simulink model "AFC_FFNN_trainbfg_15_15_15_15_Nor_July_15_RepFast"  (R2021a)
settings: Solver=ode15s  StartTime=0.0  StopTime=T  MaxStep=.01  RelTol=1e-3
undefined symbols (not defined in the file): AF_sensor_tol, fault_time, fuel_inj_tol, kappa_tol, MAF_sensor_tol, patch_sig, pump_tol, safe_patch_sig, sw, tau_ww_tol, x_gain, x_offset, y_gain, y_offset
libraries: neural x66, simulink x3
(part 3 of 3)

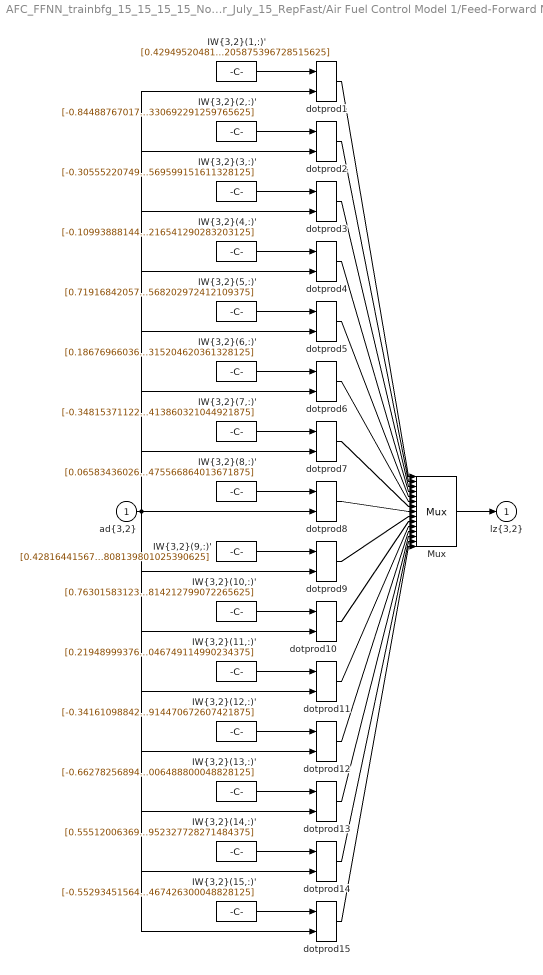
== system AFC_FFNN_trainbfg_15_15_15_15_Nor_July_15_RepFast/Air Fuel Control Model 1/Feed-Forward Neural Network/Layer 3/LW{3,2} ==
  "ad{3,2}" : Inport  PortDimensions=15
      mask Display: e = 0.06;c1 = [120 230 180]/255;c2 = ([120 230 180]+0)/(256+128);c3 = ([120 230 180]+128)/(256+128);patch([0 1 1 0],[0 0 1 1],c1);patch([0 1 1 1-e 1-e 0+e],[0 0 1 1-e 0+e 0+e],c2);patch([0 0 1 1-e 0+e 0+e],[0 1 1 1-e 1-e 0+e],c3);plot([0 1 1 0 0],[0 0 1 1 0]);
  "IW{3,2}(1,:)'" : Constant  Value=[0.4294952048164033531207905980409123003482818603515625;-0.612678315643889082053874517441727221012115478515625;-0.41663875275807360498703246776130981743335723876953125;-0.5383112997877292915660518701770342886447906494140625;-0.493758505920776968878271873109042644500732421875;-0.4693349103558774881861381800263188779354095458984375;0.2066025308635509871724167396678240038454532623291015625;0.465960500926316967262863499854574911296367645263671875;0.7996983840137072974130205693654716014862060546875;-0.01536163101939420905228672609155182726681232452392578125;-0.4735079014873659897233437732211314141750335693359375;0.048185810994904536286309593151599983684718608856201171875;0.6244275337507332324094022624194622039794921875;-0.11131049593420443144520248779372195713222026824951171875;0.63703528847606760709965101341367699205875396728515625]
      mask Display: e = 0.06;c1 = [120 150 230]/255;c2 = ([120 150 230]+0)/383;c3 = ([120 150 230]+128)/383;patch([0 1 1 0],[0 0 1 1],c1);patch([0 1 1 1-e 1-e 0+e],[0 0 1 1-e 0+e 0+e],c2);patch([0 0 1 1-e 0+e 0+e],[0 1 1 1-e 1-e 0+e],c3);plot([0 1 1 0 0],[0 0 1 1 0]);disp('weights');
  "IW{3,2}(10,:)'" : Constant  Value=[0.7630158312346824178717952236183919012546539306640625;0.1984316808513547913950247902903356589376926422119140625;-0.82423007976842577182452487249975092709064483642578125;1.0226211205456607888919506876845844089984893798828125;0.739625288102554900859786357614211738109588623046875;-0.2417860871958233681677796766962273977696895599365234375;0.44995290604095483644186970195733010768890380859375;0.9976633534078038767489715610281564295291900634765625;0.26713856145543279918541657025343738496303558349609375;-0.32276591319424319248554411387885920703411102294921875;-0.0162040947031620863327816550736315548419952392578125;0.917692798491053896015046120737679302692413330078125;-0.89634757541265097646743242876254953444004058837890625;-0.07517365498519591737736078584930510260164737701416015625;0.635019639107901046060078442678786814212799072265625]
      mask Display: e = 0.06;c1 = [120 150 230]/255;c2 = ([120 150 230]+0)/383;c3 = ([120 150 230]+128)/383;patch([0 1 1 0],[0 0 1 1],c1);patch([0 1 1 1-e 1-e 0+e],[0 0 1 1-e 0+e 0+e],c2);patch([0 0 1 1-e 0+e 0+e],[0 1 1 1-e 1-e 0+e],c3);plot([0 1 1 0 0],[0 0 1 1 0]);disp('weights');
  "IW{3,2}(11,:)'" : Constant  Value=[0.219489993767322477680181691539473831653594970703125;-0.052080718123408677178165504528806195594370365142822265625;0.8628210117321575278737100234138779342174530029296875;-0.35442212669388017953764347112155519425868988037109375;-0.1590347864723649085050283247255720198154449462890625;1.363795369435750526321271536289714276790618896484375;-0.001054289977101671195447440965153873548842966556549072265625;0.36148378499434208332985463130171410739421844482421875;0.0823384967626836772325304991682060062885284423828125;-0.238644865874834188890218911183183081448078155517578125;0.0105659440395431403203474474139511585235595703125;-0.61124435721228354001510751913883723318576812744140625;1.2260791554399050884427424534806050360202789306640625;-0.27460477604993294153956640002434141933917999267578125;-0.1981978971777476894455816136542125605046749114990234375]
      mask Display: e = 0.06;c1 = [120 150 230]/255;c2 = ([120 150 230]+0)/383;c3 = ([120 150 230]+128)/383;patch([0 1 1 0],[0 0 1 1],c1);patch([0 1 1 1-e 1-e 0+e],[0 0 1 1-e 0+e 0+e],c2);patch([0 0 1 1-e 0+e 0+e],[0 1 1 1-e 1-e 0+e],c3);plot([0 1 1 0 0],[0 0 1 1 0]);disp('weights');
  "IW{3,2}(12,:)'" : Constant  Value=[-0.341610988428120432303103370941244065761566162109375;-0.00116667452464628662416046278593739771167747676372528076171875;0.20784158680182518441625916238990612328052520751953125;-0.07459817549295848226886818110870081000030040740966796875;0.629697204521345810235288809053599834442138671875;0.8865714109056013203513657572329975664615631103515625;-0.321810848017774986384864632782409898936748504638671875;0.432273916709559336002399732024059630930423736572265625;0.379607625872108778164459863546653650701045989990234375;0.57171490814849323935931124651688151061534881591796875;0.1472744754105674847011187011958099901676177978515625;0.460402115286616286926602015228127129375934600830078125;0.10741000111703445651922805836875340901315212249755859375;-0.9041271141678794975860000704415142536163330078125;-0.443306183838275635888948045248980633914470672607421875]
      mask Display: e = 0.06;c1 = [120 150 230]/255;c2 = ([120 150 230]+0)/383;c3 = ([120 150 230]+128)/383;patch([0 1 1 0],[0 0 1 1],c1);patch([0 1 1 1-e 1-e 0+e],[0 0 1 1-e 0+e 0+e],c2);patch([0 0 1 1-e 0+e 0+e],[0 1 1 1-e 1-e 0+e],c3);plot([0 1 1 0 0],[0 0 1 1 0]);disp('weights');
  "IW{3,2}(13,:)'" : Constant  Value=[-0.66278256894771292451196131878532469272613525390625;-1.672291331705338279789430089294910430908203125;-0.38098498454672913293705960313673131167888641357421875;0.2983177358270283630048425038694404065608978271484375;-0.9202199705157365627883336856029927730560302734375;-1.6388389412374377851477902368060313165187835693359375;-0.7448345748382845243895644671283662319183349609375;0.77021932698641226711089302625623531639575958251953125;-1.2315395326944422738080220369738526642322540283203125;0.1128863476450611968981974087000708095729351043701171875;-0.8513836971448534018946929791127331554889678955078125;-1.0258859877296082618869377256487496197223663330078125;-1.39387245449321373058637618669308722019195556640625;-0.8687091691382116120934142600162886083126068115234375;-0.7700777924421189357673256381531246006488800048828125]
      mask Display: e = 0.06;c1 = [120 150 230]/255;c2 = ([120 150 230]+0)/383;c3 = ([120 150 230]+128)/383;patch([0 1 1 0],[0 0 1 1],c1);patch([0 1 1 1-e 1-e 0+e],[0 0 1 1-e 0+e 0+e],c2);patch([0 0 1 1-e 0+e 0+e],[0 1 1 1-e 1-e 0+e],c3);plot([0 1 1 0 0],[0 0 1 1 0]);disp('weights');
  "IW{3,2}(14,:)'" : Constant  Value=[0.555120063696358467808522618724964559078216552734375;-0.09894607580444551853116053052872302941977977752685546875;0.305756013218437872058785842455108650028705596923828125;-0.2069757069841939578491718521036091260612010955810546875;0.5236794338292234396448066036100499331951141357421875;0.781578562966814160972717218101024627685546875;0.925770941019874893385122049949131906032562255859375;-0.226360645757738065952935357927344739437103271484375;-0.62344387744347640190056836217991076409816741943359375;-0.54223723805426360389247975035686977207660675048828125;-0.3542426822873754321818751122918911278247833251953125;-0.10062609396851908416525844813804724253714084625244140625;-0.60891512989643270525874640952679328620433807373046875;-0.053775078503994037937285810357934678904712200164794921875;-0.7076681573893226495641783913015387952327728271484375]
      mask Display: e = 0.06;c1 = [120 150 230]/255;c2 = ([120 150 230]+0)/383;c3 = ([120 150 230]+128)/383;patch([0 1 1 0],[0 0 1 1],c1);patch([0 1 1 1-e 1-e 0+e],[0 0 1 1-e 0+e 0+e],c2);patch([0 0 1 1-e 0+e 0+e],[0 1 1 1-e 1-e 0+e],c3);plot([0 1 1 0 0],[0 0 1 1 0]);disp('weights');
  "IW{3,2}(15,:)'" : Constant  Value=[-0.552934515642912405297693112515844404697418212890625;-0.30075123633298284087089768945588730275630950927734375;-0.08501069722579314424937280136873596347868442535400390625;0.72562881316305161139013080173754133284091949462890625;-0.079368032880180461319241658202372491359710693359375;-0.7423600633093923040206618679803796112537384033203125;0.408580117977064116718821651375037617981433868408203125;-0.6116357762143371790131141096935607492923736572265625;0.08264039362662288501493179637691355310380458831787109375;0.347506445741584124586864845696254633367061614990234375;-0.9886562132901974830900826418655924499034881591796875;0.94918588506836709672853658048552460968494415283203125;1.0474680392741293477598674144246615469455718994140625;0.53384758038892687892484900658018887042999267578125;-0.2372585876275876970442624269708176143467426300048828125]
      mask Display: e = 0.06;c1 = [120 150 230]/255;c2 = ([120 150 230]+0)/383;c3 = ([120 150 230]+128)/383;patch([0 1 1 0],[0 0 1 1],c1);patch([0 1 1 1-e 1-e 0+e],[0 0 1 1-e 0+e 0+e],c2);patch([0 0 1 1-e 0+e 0+e],[0 1 1 1-e 1-e 0+e],c3);plot([0 1 1 0 0],[0 0 1 1 0]);disp('weights');
  "IW{3,2}(2,:)'" : Constant  Value=[-0.8448876701768590624652688347850926220417022705078125;-0.0538388952155621769435356327448971569538116455078125;-0.2690932818904168133400389706366695463657379150390625;-0.98017730775724920544433871327782981097698211669921875;-0.37904000714715646580543761956505477428436279296875;-0.31094857201915060418428993216366507112979888916015625;0.219769365539062899728151023737154901027679443359375;-0.5910279837821719173263090851833112537860870361328125;-0.6862175631530516017875243051094003021717071533203125;-0.6523710301420024837426581143517978489398956298828125;-0.34206029681594340985384405939839780330657958984375;0.239587834758158368941849403199739754199981689453125;0.6623164964936882892487801655079238116741180419921875;0.6427690120268698681371688508079387247562408447265625;-0.81383550246944358352862991523579694330692291259765625]
      mask Display: e = 0.06;c1 = [120 150 230]/255;c2 = ([120 150 230]+0)/383;c3 = ([120 150 230]+128)/383;patch([0 1 1 0],[0 0 1 1],c1);patch([0 1 1 1-e 1-e 0+e],[0 0 1 1-e 0+e 0+e],c2);patch([0 0 1 1-e 0+e 0+e],[0 1 1 1-e 1-e 0+e],c3);plot([0 1 1 0 0],[0 0 1 1 0]);disp('weights');
  "IW{3,2}(3,:)'" : Constant  Value=[-0.3055522074982641722584730814560316503047943115234375;0.5665869649025629950500615450437180697917938232421875;0.071199336634411081181639247006387449800968170166015625;0.288339577238945654613644364872016012668609619140625;0.4106526758379249741892635938711464405059814453125;0.385876628268256360865251508585060946643352508544921875;0.0914900373172624625794924213550984859466552734375;-0.36248110666585464656463955179788172245025634765625;0.09184886789510234017530621031255577690899372100830078125;0.0193957862645101654364143684006194234825670719146728515625;0.7238374758794805519102055768598802387714385986328125;0.3132733782825980473063509634812362492084503173828125;-0.83750985046541781553486316624912433326244354248046875;0.604369831840676940970524810836650431156158447265625;0.80651036891984262400256966429878957569599151611328125]
      mask Display: e = 0.06;c1 = [120 150 230]/255;c2 = ([120 150 230]+0)/383;c3 = ([120 150 230]+128)/383;patch([0 1 1 0],[0 0 1 1],c1);patch([0 1 1 1-e 1-e 0+e],[0 0 1 1-e 0+e 0+e],c2);patch([0 0 1 1-e 0+e 0+e],[0 1 1 1-e 1-e 0+e],c3);plot([0 1 1 0 0],[0 0 1 1 0]);disp('weights');
  "IW{3,2}(4,:)'" : Constant  Value=[-0.1099388814495494415268694865517318248748779296875;0.6187779335822465309746576167526654899120330810546875;0.516841841257460021807901284773834049701690673828125;-0.524964717876703179655351050314493477344512939453125;-0.362800002813841171445119471172802150249481201171875;-0.8831515396491536051826187758706510066986083984375;-0.4767342557674947300938583794049918651580810546875;0.2933585055759546644793545056018047034740447998046875;0.0045669865725361802333281957544386386871337890625;-0.0906953734773459085971580861951224505901336669921875;0.706787173330524876035951820085756480693817138671875;-0.5622356034924251844131504185497760772705078125;0.348462004036084405100837102509103715419769287109375;-0.0357165571439550522114814157248474657535552978515625;-0.1130256756824661312776925115031190216541290283203125]
      mask Display: e = 0.06;c1 = [120 150 230]/255;c2 = ([120 150 230]+0)/383;c3 = ([120 150 230]+128)/383;patch([0 1 1 0],[0 0 1 1],c1);patch([0 1 1 1-e 1-e 0+e],[0 0 1 1-e 0+e 0+e],c2);patch([0 0 1 1-e 0+e 0+e],[0 1 1 1-e 1-e 0+e],c3);plot([0 1 1 0 0],[0 0 1 1 0]);disp('weights');
  "IW{3,2}(5,:)'" : Constant  Value=[0.719168420574110456300331861712038516998291015625;0.0847737795487171208463905713870190083980560302734375;-0.141553298693671780750236166568356566131114959716796875;0.6788606635025420388274142169393599033355712890625;0.8932262043684249253061580020585097372531890869140625;-0.241966142969885555924491882251459173858165740966796875;-0.739255956912197031982714179321192204952239990234375;-0.7400967432848950533497145443107001483440399169921875;-0.2422206485527137742597147962442249990999698638916015625;0.5005674876542745010965518304146826267242431640625;-0.9594575603270742991668385002412833273410797119140625;0.197719552715467539183435974337044171988964080810546875;0.3366654479273407662986983268638141453266143798828125;-0.13031606394009942473388719008653424680233001708984375;0.73395107780940482822273907004273496568202972412109375]
      mask Display: e = 0.06;c1 = [120 150 230]/255;c2 = ([120 150 230]+0)/383;c3 = ([120 150 230]+128)/383;patch([0 1 1 0],[0 0 1 1],c1);patch([0 1 1 1-e 1-e 0+e],[0 0 1 1-e 0+e 0+e],c2);patch([0 0 1 1-e 0+e 0+e],[0 1 1 1-e 1-e 0+e],c3);plot([0 1 1 0 0],[0 0 1 1 0]);disp('weights');
  "IW{3,2}(6,:)'" : Constant  Value=[0.186769660362741785064599753241054713726043701171875;0.5620259810922336729532844401546753942966461181640625;-0.11959347594884039978069267817772924900054931640625;0.2975256040824234560204786248505115509033203125;-0.47897995742988808132167832809500396251678466796875;-0.1724617171978507224050503054968430660665035247802734375;-0.312929225364951768550980659711058251559734344482421875;0.71983954572869823795855381831643171608448028564453125;0.4738927604266383042386223678477108478546142578125;0.59121953726546350171844323995173908770084381103515625;-0.132711710780250680130620821728371083736419677734375;0.88317009485144382097132620401680469512939453125;-0.390049186299380734599395736950100399553775787353515625;0.2089508793613176484971205582041875459253787994384765625;-0.7894884252939420310468676689197309315204620361328125]
      mask Display: e = 0.06;c1 = [120 150 230]/255;c2 = ([120 150 230]+0)/383;c3 = ([120 150 230]+128)/383;patch([0 1 1 0],[0 0 1 1],c1);patch([0 1 1 1-e 1-e 0+e],[0 0 1 1-e 0+e 0+e],c2);patch([0 0 1 1-e 0+e 0+e],[0 1 1 1-e 1-e 0+e],c3);plot([0 1 1 0 0],[0 0 1 1 0]);disp('weights');
  "IW{3,2}(7,:)'" : Constant  Value=[-0.34815371122304039630535044125281274318695068359375;-0.2320934798606277826849009215948171913623809814453125;-0.8177263878639149385918472034973092377185821533203125;-0.4004659264562528964148668819689191877841949462890625;0.9852052407892359919827640624134801328182220458984375;-0.8790860570702019316513542435131967067718505859375;-0.7520229089538961186889309828984551131725311279296875;-0.486310433836135036500536443782038986682891845703125;0.0804089058620609531402578795677982270717620849609375;0.1939113091998303506358070080750621855258941650390625;-0.5694334409514791861539606543374247848987579345703125;0.041020374400621673061095862067304551601409912109375;-0.63187403134157360540257286629639565944671630859375;0.406940419921116625090462548541836440563201904296875;-0.638383341242963364692286631907336413860321044921875]
      mask Display: e = 0.06;c1 = [120 150 230]/255;c2 = ([120 150 230]+0)/383;c3 = ([120 150 230]+128)/383;patch([0 1 1 0],[0 0 1 1],c1);patch([0 1 1 1-e 1-e 0+e],[0 0 1 1-e 0+e 0+e],c2);patch([0 0 1 1-e 0+e 0+e],[0 1 1 1-e 1-e 0+e],c3);plot([0 1 1 0 0],[0 0 1 1 0]);disp('weights');
  "IW{3,2}(8,:)'" : Constant  Value=[0.065834360268933966864324247580952942371368408203125;-0.8587358519232417553013192446087487041950225830078125;-0.3757028777741744374196741773630492389202117919921875;0.387381441438808149513306489097885787487030029296875;-0.7623660854903249184388869252870790660381317138671875;0.578378113811186977955003385432064533233642578125;0.92802774539068533243835190660320222377777099609375;0.9315222419608926163192563763004727661609649658203125;-0.4453573868828100135175418472499586641788482666015625;-0.3239075921512151179371130638173781335353851318359375;-0.543094684532615445959891076199710369110107421875;0.265181424379623109643944189883768558502197265625;-0.8358578306212993691559631770360283553600311279296875;0.2872139959247246299156586246681399643421173095703125;0.0983004378392535738129254241357557475566864013671875]
      mask Display: e = 0.06;c1 = [120 150 230]/255;c2 = ([120 150 230]+0)/383;c3 = ([120 150 230]+128)/383;patch([0 1 1 0],[0 0 1 1],c1);patch([0 1 1 1-e 1-e 0+e],[0 0 1 1-e 0+e 0+e],c2);patch([0 0 1 1-e 0+e 0+e],[0 1 1 1-e 1-e 0+e],c3);plot([0 1 1 0 0],[0 0 1 1 0]);disp('weights');
  "IW{3,2}(9,:)'" : Constant  Value=[0.4281644156755806118752616384881548583507537841796875;-0.91161616821853908021466850186698138713836669921875;0.069575991587280672234783196472562849521636962890625;-0.6533917177043384594270492016221396625041961669921875;-0.919023562922785419715410171193070709705352783203125;-0.8818394943501479676939425189630128443241119384765625;0.244561023694448209653273806907236576080322265625;0.00809787728502708858968617278151214122772216796875;0.4934701959927141334816269591101445257663726806640625;0.1884537709115605697007822527666576206684112548828125;0.4950349159460785131159354932606220245361328125;-0.2472134903970317765242725727148354053497314453125;-0.026650106766705761174307554028928279876708984375;0.211677611937319820611946852295659482479095458984375;-0.474173165212278036051429808139801025390625]
      mask Display: e = 0.06;c1 = [120 150 230]/255;c2 = ([120 150 230]+0)/383;c3 = ([120 150 230]+128)/383;patch([0 1 1 0],[0 0 1 1],c1);patch([0 1 1 1-e 1-e 0+e],[0 0 1 1-e 0+e 0+e],c2);patch([0 0 1 1-e 0+e 0+e],[0 1 1 1-e 1-e 0+e],c3);plot([0 1 1 0 0],[0 0 1 1 0]);disp('weights');
  Mux : Mux  Inputs=15
      mask Display: e = 0.06;c1 = [120 150 230]/255;c2 = ([120 150 230]+0)/383;c3 = ([120 150 230]+128)/383;patch([0 1 1 0],[0 0 1 1],c1);patch([0 1 1 1-e 1-e 0+e],[0 0 1 1-e 0+e 0+e],c2);patch([0 0 1 1-e 0+e 0+e],[0 1 1 1-e 1-e 0+e],c3);plot([0 1 1 0 0],[0 0 1 1 0]);disp('Mux');
  dotprod{1..15} (15 alike) : neural/Weight Functions/dotprod
  "lz{3,2}" : Outport
      mask Display: e = 0.06;c1 = [120 230 180]/255;c2 = ([120 230 180]+0)/(256+128);c3 = ([120 230 180]+128)/(256+128);patch([0 1 1 0],[0 0 1 1],c1);patch([0 1 1 1-e 1-e 0+e],[0 0 1 1-e 0+e 0+e],c2);patch([0 0 1 1-e 0+e 0+e],[0 1 1 1-e 1-e 0+e],c3);plot([0 1 1 0 0],[0 0 1 1 0]);
  wires:
  Mux/1 -> "lz{3,2}"/1
  dotprod15/1 -> Mux/15
  "IW{3,2}(15,:)'"/1 -> dotprod15/1
  dotprod14/1 -> Mux/14
  "IW{3,2}(14,:)'"/1 -> dotprod14/1
  dotprod13/1 -> Mux/13
  "IW{3,2}(13,:)'"/1 -> dotprod13/1
  dotprod12/1 -> Mux/12
  "IW{3,2}(12,:)'"/1 -> dotprod12/1
  dotprod11/1 -> Mux/11
  "IW{3,2}(11,:)'"/1 -> dotprod11/1
  dotprod10/1 -> Mux/10
  "IW{3,2}(10,:)'"/1 -> dotprod10/1
  dotprod9/1 -> Mux/9
  "IW{3,2}(9,:)'"/1 -> dotprod9/1
  dotprod8/1 -> Mux/8
  "IW{3,2}(8,:)'"/1 -> dotprod8/1
  dotprod7/1 -> Mux/7
  "IW{3,2}(7,:)'"/1 -> dotprod7/1
  dotprod6/1 -> Mux/6
  "IW{3,2}(6,:)'"/1 -> dotprod6/1
  dotprod5/1 -> Mux/5
  "IW{3,2}(5,:)'"/1 -> dotprod5/1
  dotprod4/1 -> Mux/4
  "IW{3,2}(4,:)'"/1 -> dotprod4/1
  dotprod3/1 -> Mux/3
  "IW{3,2}(3,:)'"/1 -> dotprod3/1
  dotprod2/1 -> Mux/2
  "IW{3,2}(2,:)'"/1 -> dotprod2/1
  dotprod1/1 -> Mux/1
  "ad{3,2}"/1 -> dotprod15/2, dotprod14/2, dotprod13/2, dotprod12/2, dotprod11/2, dotprod10/2, dotprod9/2, dotprod8/2, dotprod7/2, dotprod6/2, dotprod5/2, dotprod4/2, dotprod3/2, dotprod2/2, dotprod1/2
  "IW{3,2}(1,:)'"/1 -> dotprod1/1

== system AFC_FFNN_trainbfg_15_15_15_15_Nor_July_15_RepFast/Air Fuel Control Model 1/Feed-Forward Neural Network/Layer 4/Delays 1 ==
  "p{4}" : Inport  PortDimensions=15
      mask Display: e = 0.06;c1 = [120 230 180]/255;c2 = ([120 230 180]+0)/(256+128);c3 = ([120 230 180]+128)/(256+128);patch([0 1 1 0],[0 0 1 1],c1);patch([0 1 1 1-e 1-e 0+e],[0 0 1 1-e 0+e 0+e],c2);patch([0 0 1 1-e 0+e 0+e],[0 1 1 1-e 1-e 0+e],c3);plot([0 1 1 0 0],[0 0 1 1 0]);
  mux : Mux  Inputs=1
      mask Display: e = 0.06;c1 = [120 150 230]/255;c2 = ([120 150 230]+0)/383;c3 = ([120 150 230]+128)/383;patch([0 1 1 0],[0 0 1 1],c1);patch([0 1 1 1-e 1-e 0+e],[0 0 1 1-e 0+e 0+e],c2);patch([0 0 1 1-e 0+e 0+e],[0 1 1 1-e 1-e 0+e],c3);plot([0 1 1 0 0],[0 0 1 1 0]);disp('Mux')
  "pd{4,3}" : Outport
      mask Display: e = 0.06;c1 = [120 230 180]/255;c2 = ([120 230 180]+0)/(256+128);c3 = ([120 230 180]+128)/(256+128);patch([0 1 1 0],[0 0 1 1],c1);patch([0 1 1 1-e 1-e 0+e],[0 0 1 1-e 0+e 0+e],c2);patch([0 0 1 1-e 0+e 0+e],[0 1 1 1-e 1-e 0+e],c3);plot([0 1 1 0 0],[0 0 1 1 0]);
  wires:
  mux/1 -> "pd{4,3}"/1
  "p{4}"/1 -> mux/1

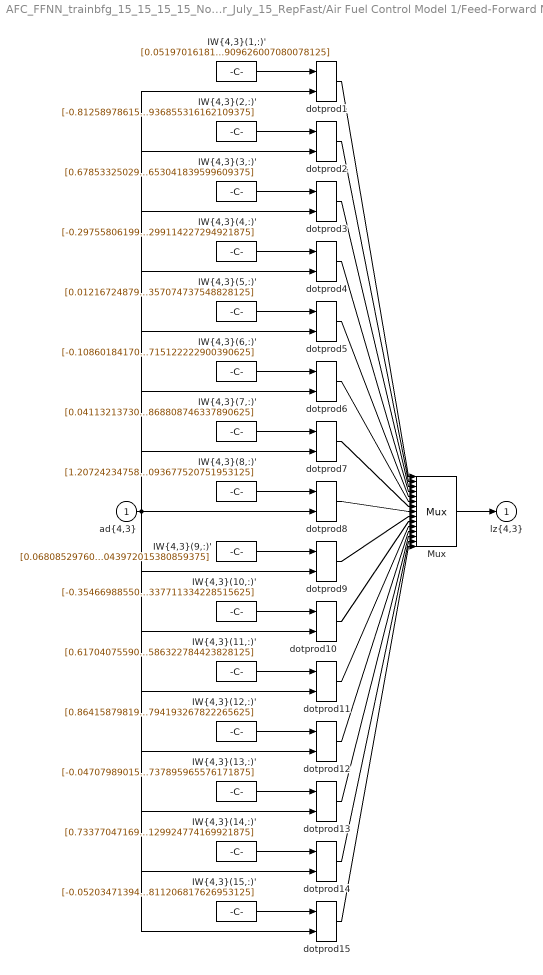
== system AFC_FFNN_trainbfg_15_15_15_15_Nor_July_15_RepFast/Air Fuel Control Model 1/Feed-Forward Neural Network/Layer 4/LW{4,3} ==
  "ad{4,3}" : Inport  PortDimensions=15
      mask Display: e = 0.06;c1 = [120 230 180]/255;c2 = ([120 230 180]+0)/(256+128);c3 = ([120 230 180]+128)/(256+128);patch([0 1 1 0],[0 0 1 1],c1);patch([0 1 1 1-e 1-e 0+e],[0 0 1 1-e 0+e 0+e],c2);patch([0 0 1 1-e 0+e 0+e],[0 1 1 1-e 1-e 0+e],c3);plot([0 1 1 0 0],[0 0 1 1 0]);
  "IW{4,3}(1,:)'" : Constant  Value=[0.051970161810708959126969830322195775806903839111328125;-0.126328957419962417674241805798374116420745849609375;0.9965377844405078899825412008794955909252166748046875;0.1675357955800376164035014880937524139881134033203125;0.404152985833085953704113535422948189079761505126953125;0.86478973592762808930700657583656720817089080810546875;0.518227264629068873347250701044686138629913330078125;0.2715980210299460129164117461186833679676055908203125;-0.651185893458846809522810872294940054416656494140625;0.319204255476944143143924748073914088308811187744140625;-0.2569115041239822261331937625072896480560302734375;0.057105623983778171226521891412630793638527393341064453125;0.1070777617804902492881780062816687859594821929931640625;-0.82642827178341027316577083183801732957363128662109375;-0.0287179233202064232433059487448190338909626007080078125]
      mask Display: e = 0.06;c1 = [120 150 230]/255;c2 = ([120 150 230]+0)/383;c3 = ([120 150 230]+128)/383;patch([0 1 1 0],[0 0 1 1],c1);patch([0 1 1 1-e 1-e 0+e],[0 0 1 1-e 0+e 0+e],c2);patch([0 0 1 1-e 0+e 0+e],[0 1 1 1-e 1-e 0+e],c3);plot([0 1 1 0 0],[0 0 1 1 0]);disp('weights');
  "IW{4,3}(10,:)'" : Constant  Value=[-0.354669885508523241579581508631235919892787933349609375;-0.77194952346326062286863134431769140064716339111328125;-0.81601175837494732689947340986691415309906005859375;0.379241236877119636261568302870728075504302978515625;-0.3569337623701613892990280874073505401611328125;-0.792692853946006525944767417968250811100006103515625;-0.14953643024327778476845196564681828022003173828125;-0.0850888851491766740053890316630713641643524169921875;-0.9650803191481467369072788642370142042636871337890625;0.405282382043266498072853210032917559146881103515625;0.49853527113881723753507912988425232470035552978515625;0.271502161657881657674806774593889713287353515625;0.3751637008352275426403821256826631724834442138671875;0.8806065157679683341740428659250028431415557861328125;-0.59715081395340219305722939679981209337711334228515625]
      mask Display: e = 0.06;c1 = [120 150 230]/255;c2 = ([120 150 230]+0)/383;c3 = ([120 150 230]+128)/383;patch([0 1 1 0],[0 0 1 1],c1);patch([0 1 1 1-e 1-e 0+e],[0 0 1 1-e 0+e 0+e],c2);patch([0 0 1 1-e 0+e 0+e],[0 1 1 1-e 1-e 0+e],c3);plot([0 1 1 0 0],[0 0 1 1 0]);disp('weights');
  "IW{4,3}(11,:)'" : Constant  Value=[0.617040755904621818217492545954883098602294921875;0.700604235086529580911474113236181437969207763671875;0.511371924663512888997729533002711832523345947265625;0.08963480551315772260068115429021418094635009765625;-0.165964035301581269710169408426736481487751007080078125;0.5031390236482307098953015156439505517482757568359375;0.6633082060229267273854247832787223160266876220703125;-0.709798207981374940089835945400409400463104248046875;0.831096977986841789487471032771281898021697998046875;-0.4122922604000514024136236912454478442668914794921875;-0.0723067339924330365619198346394114196300506591796875;-0.376003397439505893107281053744372911751270294189453125;0.1695995889177781823509150171958026476204395294189453125;0.90183804417739477088389321579597890377044677734375;-1.10240234673867565362570530851371586322784423828125]
      mask Display: e = 0.06;c1 = [120 150 230]/255;c2 = ([120 150 230]+0)/383;c3 = ([120 150 230]+128)/383;patch([0 1 1 0],[0 0 1 1],c1);patch([0 1 1 1-e 1-e 0+e],[0 0 1 1-e 0+e 0+e],c2);patch([0 0 1 1-e 0+e 0+e],[0 1 1 1-e 1-e 0+e],c3);plot([0 1 1 0 0],[0 0 1 1 0]);disp('weights');
  "IW{4,3}(12,:)'" : Constant  Value=[0.86415879819654961568886619716067798435688018798828125;0.1203834479508809618408804453792981803417205810546875;0.133982984467660326544091731193475425243377685546875;-0.0193712548926814331906598454224877059459686279296875;-0.1402303904538838852378290766864665783941745758056640625;1.0897626729878930884609644635929726064205169677734375;0.67839995473971459460926780593581497669219970703125;-0.7508734295524204238603260819218121469020843505859375;0.0334637355957545512552542277262546122074127197265625;0.87659168440380941245138046724605374038219451904296875;-0.980282012415287784534712045569904148578643798828125;0.8080715194356573594092196799465455114841461181640625;-0.76798820148797342088897721623652614653110504150390625;-0.313277713257333612073551876164856366813182830810546875;0.35824559123448074249296269044862128794193267822265625]
      mask Display: e = 0.06;c1 = [120 150 230]/255;c2 = ([120 150 230]+0)/383;c3 = ([120 150 230]+128)/383;patch([0 1 1 0],[0 0 1 1],c1);patch([0 1 1 1-e 1-e 0+e],[0 0 1 1-e 0+e 0+e],c2);patch([0 0 1 1-e 0+e 0+e],[0 1 1 1-e 1-e 0+e],c3);plot([0 1 1 0 0],[0 0 1 1 0]);disp('weights');
  "IW{4,3}(13,:)'" : Constant  Value=[-0.04707989015845824576356193347237422131001949310302734375;-0.74905307149987765402698869365849532186985015869140625;0.5757676864781038350571407136158086359500885009765625;0.71306953158993646724184145568870007991790771484375;-0.5913842257991495099389567258185707032680511474609375;-0.37587419944126232440595458683674223721027374267578125;-0.336733940480412829998613233328796923160552978515625;-0.004068794637174466544138340395875275135040283203125;0.0693886439127837650886476694722659885883331298828125;0.05129647141780004082622923533563152886927127838134765625;-0.0307644877411348029172533102837405749596655368804931640625;-0.334572257247817306247128499308018945157527923583984375;0.2420501582242300664393752640535240061581134796142578125;-0.77793738892486985481156125388224609196186065673828125;1.190993380582610949858235471765510737895965576171875]
      mask Display: e = 0.06;c1 = [120 150 230]/255;c2 = ([120 150 230]+0)/383;c3 = ([120 150 230]+128)/383;patch([0 1 1 0],[0 0 1 1],c1);patch([0 1 1 1-e 1-e 0+e],[0 0 1 1-e 0+e 0+e],c2);patch([0 0 1 1-e 0+e 0+e],[0 1 1 1-e 1-e 0+e],c3);plot([0 1 1 0 0],[0 0 1 1 0]);disp('weights');
  "IW{4,3}(14,:)'" : Constant  Value=[0.73377047169310072316505966227850876748561859130859375;0.59318557483826050980013633306953124701976776123046875;0.97198033802115357815409879549406468868255615234375;-0.6828295214165047699594879304640926420688629150390625;-0.727325596267671681260935656609944999217987060546875;-0.007302479939687057074182430227438089787028729915618896484375;-0.74322529652487201445865139248780906200408935546875;0.2139264100071509577816186720156110823154449462890625;0.7427593592867605121199403583887033164501190185546875;-0.6586018858724387303738012633402831852436065673828125;-0.1654446667255996816781049574274220503866672515869140625;0.46870267206282634209202342390199191868305206298828125;-0.2075915391437903878557591497155954129993915557861328125;0.271907738610796367861865974191459827125072479248046875;-0.1551503657733785679351257158486987464129924774169921875]
      mask Display: e = 0.06;c1 = [120 150 230]/255;c2 = ([120 150 230]+0)/383;c3 = ([120 150 230]+128)/383;patch([0 1 1 0],[0 0 1 1],c1);patch([0 1 1 1-e 1-e 0+e],[0 0 1 1-e 0+e 0+e],c2);patch([0 0 1 1-e 0+e 0+e],[0 1 1 1-e 1-e 0+e],c3);plot([0 1 1 0 0],[0 0 1 1 0]);disp('weights');
  "IW{4,3}(15,:)'" : Constant  Value=[-0.052034713940864042724943061557496548630297183990478515625;0.7331140203109469677400511500309221446514129638671875;0.134145500728414412972000491208746097981929779052734375;0.14154267621595284509794510086067020893096923828125;0.2930468609746219588174653836176730692386627197265625;0.4199159074445060202407375982147641479969024658203125;-0.93186243047858141608230653218924999237060546875;0.04270707824443764621946684201247990131378173828125;0.350319910837068260178739365073852241039276123046875;-0.342224755301396121875967537562246434390544891357421875;0.12252060779661462508460800790999201126396656036376953125;0.253549817145111544558488958500674925744533538818359375;0.89990162781650495649188314928323961794376373291015625;0.9157133079961587984740845058695413172245025634765625;-0.55171023855309730965501557875541038811206817626953125]
      mask Display: e = 0.06;c1 = [120 150 230]/255;c2 = ([120 150 230]+0)/383;c3 = ([120 150 230]+128)/383;patch([0 1 1 0],[0 0 1 1],c1);patch([0 1 1 1-e 1-e 0+e],[0 0 1 1-e 0+e 0+e],c2);patch([0 0 1 1-e 0+e 0+e],[0 1 1 1-e 1-e 0+e],c3);plot([0 1 1 0 0],[0 0 1 1 0]);disp('weights');
  "IW{4,3}(2,:)'" : Constant  Value=[-0.8125897861595652305055637043551541864871978759765625;0.6696301702838931557693058493896387517452239990234375;0.0494682777685733210404350757016800343990325927734375;0.817877680294583964126786668202839791774749755859375;0.148708664585286864934232653467915952205657958984375;-0.1140448432503557985029374322039075195789337158203125;0.2540073049131656990340388801996596157550811767578125;-0.0952829278543816382551767674158327281475067138671875;-0.869787452715599318509021031786687672138214111328125;0.0628607068926652079454697741311974823474884033203125;-0.99548355810059963033609164995141327381134033203125;0.7449122353879769065088112256489694118499755859375;0.54699886858855517601796236704103648662567138671875;-0.6575546792262390027872243081219494342803955078125;-0.1118978718546799200339592061936855316162109375]
      mask Display: e = 0.06;c1 = [120 150 230]/255;c2 = ([120 150 230]+0)/383;c3 = ([120 150 230]+128)/383;patch([0 1 1 0],[0 0 1 1],c1);patch([0 1 1 1-e 1-e 0+e],[0 0 1 1-e 0+e 0+e],c2);patch([0 0 1 1-e 0+e 0+e],[0 1 1 1-e 1-e 0+e],c3);plot([0 1 1 0 0],[0 0 1 1 0]);disp('weights');
  "IW{4,3}(3,:)'" : Constant  Value=[0.67853325029204014651185161710600368678569793701171875;0.649225618879884169842853225418366491794586181640625;0.0244182303058833767572810558021956239826977252960205078125;0.91905635318846368164713567239232361316680908203125;0.0660607060368446907805406453917385078966617584228515625;-0.11251524592039625904948962897833553142845630645751953125;0.0515896481136202122996792240883223712444305419921875;-0.5706344744726050688399254795513115823268890380859375;0.543627018010135909520386121585033833980560302734375;-0.718405788341949236297523384564556181430816650390625;0.072829230863325822298293132917024195194244384765625;1.1098893041941300108277346225804649293422698974609375;-0.6268628150142021571156192294438369572162628173828125;0.64965362929718917239796383000793866813182830810546875;0.24955078029045585363832060465938411653041839599609375]
      mask Display: e = 0.06;c1 = [120 150 230]/255;c2 = ([120 150 230]+0)/383;c3 = ([120 150 230]+128)/383;patch([0 1 1 0],[0 0 1 1],c1);patch([0 1 1 1-e 1-e 0+e],[0 0 1 1-e 0+e 0+e],c2);patch([0 0 1 1-e 0+e 0+e],[0 1 1 1-e 1-e 0+e],c3);plot([0 1 1 0 0],[0 0 1 1 0]);disp('weights');
  "IW{4,3}(4,:)'" : Constant  Value=[-0.2975580619978703822425813996233046054840087890625;0.216290439667084388730700084124691784381866455078125;-0.532417130550156603163713953108526766300201416015625;-0.9093614745271327848286091466434299945831298828125;-0.4789695686043524691655193237238563597202301025390625;-0.2897506116045913682199852701160125434398651123046875;-0.09180504603758521398049197159707546234130859375;0.0106020674426960948011355867492966353893280029296875;-0.661658236974961067033973449724726378917694091796875;0.659602628583194405820222527836449444293975830078125;-0.1565907405649149541915221561794169247150421142578125;0.1760495719019183891163038424565456807613372802734375;-0.4251169390202733655570455084671266376972198486328125;-0.2251245296180972577104739684727974236011505126953125;-0.4908767677254395334074388301814906299114227294921875]
      mask Display: e = 0.06;c1 = [120 150 230]/255;c2 = ([120 150 230]+0)/383;c3 = ([120 150 230]+128)/383;patch([0 1 1 0],[0 0 1 1],c1);patch([0 1 1 1-e 1-e 0+e],[0 0 1 1-e 0+e 0+e],c2);patch([0 0 1 1-e 0+e 0+e],[0 1 1 1-e 1-e 0+e],c3);plot([0 1 1 0 0],[0 0 1 1 0]);disp('weights');
  "IW{4,3}(5,:)'" : Constant  Value=[0.0121672487908398678502219780739324050955474376678466796875;-0.279291635237711555195261325934552587568759918212890625;0.39580478815836916961501401601708494126796722412109375;-0.41888196527845256156297182315029203891754150390625;0.96026476375696512288726580663933418691158294677734375;-0.07705788414508407679903712050872854888439178466796875;-0.7369962098884264012355060913250781595706939697265625;-0.641380277290782174759442568756639957427978515625;-0.1470570579484429263317224467755295336246490478515625;-0.552357426018287522850869208923541009426116943359375;0.5426753535136719097664581568096764385700225830078125;-0.6534036514741854428933720555505715310573577880859375;0.8952196061710460117666343649034388363361358642578125;-0.71648872638311933425114830242819152772426605224609375;1.101038667785545488442267014761455357074737548828125]
      mask Display: e = 0.06;c1 = [120 150 230]/255;c2 = ([120 150 230]+0)/383;c3 = ([120 150 230]+128)/383;patch([0 1 1 0],[0 0 1 1],c1);patch([0 1 1 1-e 1-e 0+e],[0 0 1 1-e 0+e 0+e],c2);patch([0 0 1 1-e 0+e 0+e],[0 1 1 1-e 1-e 0+e],c3);plot([0 1 1 0 0],[0 0 1 1 0]);disp('weights');
  "IW{4,3}(6,:)'" : Constant  Value=[-0.10860184170805009529203744023106992244720458984375;0.0194190021120725919701044404064305126667022705078125;0.7664594013744976397362052011885680258274078369140625;-0.0669174495247097933514623946393840014934539794921875;-0.69434533003424991903784757596440613269805908203125;-0.8237276518362877109069586367695592343807220458984375;0.2052424366817493517345383224892430007457733154296875;-0.252655580676456548161468163016252219676971435546875;0.66723256757870075261962483637034893035888671875;0.957094387199472595995075607788749039173126220703125;-0.3538932796519895784825848750188015401363372802734375;-0.7059302300365530857817475407500751316547393798828125;-0.8348335978485235120416518839192576706409454345703125;-0.00859368877235322514707149821333587169647216796875;-0.1199812481452335877207815428846515715122222900390625]
      mask Display: e = 0.06;c1 = [120 150 230]/255;c2 = ([120 150 230]+0)/383;c3 = ([120 150 230]+128)/383;patch([0 1 1 0],[0 0 1 1],c1);patch([0 1 1 1-e 1-e 0+e],[0 0 1 1-e 0+e 0+e],c2);patch([0 0 1 1-e 0+e 0+e],[0 1 1 1-e 1-e 0+e],c3);plot([0 1 1 0 0],[0 0 1 1 0]);disp('weights');
  "IW{4,3}(7,:)'" : Constant  Value=[0.041132137300131328683239217980371904559433460235595703125;-0.8170410050061052142922335406183265149593353271484375;0.880640458053120855907991426647640764713287353515625;-0.8672502897025411439102526856004260480403900146484375;0.375021567196341221173128133159480057656764984130859375;0.74060605087412023639359404114657081663608551025390625;0.208223727655667989466792278108187019824981689453125;0.4991232146158661731050187881919555366039276123046875;0.8040042399321531974010213161818683147430419921875;-0.9287241362211251516356469437596388161182403564453125;-0.2369142647526545075731263523266534321010112762451171875;-0.381204863194875620546753225426073186099529266357421875;-0.8032444535196681112410033165360800921916961669921875;0.3691943099448593557099229656159877777099609375;0.0186137077896842174917768630848513566888868808746337890625]
      mask Display: e = 0.06;c1 = [120 150 230]/255;c2 = ([120 150 230]+0)/383;c3 = ([120 150 230]+128)/383;patch([0 1 1 0],[0 0 1 1],c1);patch([0 1 1 1-e 1-e 0+e],[0 0 1 1-e 0+e 0+e],c2);patch([0 0 1 1-e 0+e 0+e],[0 1 1 1-e 1-e 0+e],c3);plot([0 1 1 0 0],[0 0 1 1 0]);disp('weights');
  "IW{4,3}(8,:)'" : Constant  Value=[1.2072423475886087107511457361397333443164825439453125;-0.11524115643226974514679028516184189356863498687744140625;0.34222553991496285075157857136218808591365814208984375;0.3645259514743426354499433728051371872425079345703125;0.339188479923518582115349317973596043884754180908203125;-0.42353456120008792229469918311224319040775299072265625;0.724771462281134315475128460093401372432708740234375;-0.6004800474653737563102140484261326491832733154296875;-0.4151526394563258559600171793135814368724822998046875;-0.338141381416675101956315074858139269053936004638671875;0.66970817401589821660223833532654680311679840087890625;-1.143557580187915423408639981062151491641998291015625;-0.2154730791377687804111218383695813827216625213623046875;0.418907292844881318227834299250389449298381805419921875;-0.23972582973012468432472132917609997093677520751953125]
      mask Display: e = 0.06;c1 = [120 150 230]/255;c2 = ([120 150 230]+0)/383;c3 = ([120 150 230]+128)/383;patch([0 1 1 0],[0 0 1 1],c1);patch([0 1 1 1-e 1-e 0+e],[0 0 1 1-e 0+e 0+e],c2);patch([0 0 1 1-e 0+e 0+e],[0 1 1 1-e 1-e 0+e],c3);plot([0 1 1 0 0],[0 0 1 1 0]);disp('weights');
  "IW{4,3}(9,:)'" : Constant  Value=[0.068085297603662386922707128178444691002368927001953125;-0.2575471222895735490254764954443089663982391357421875;-0.59973830245885439982345133103081025183200836181640625;0.77825576456782386003396823070943355560302734375;0.2305592100961315893403735799438436515629291534423828125;-0.57777072238661719705277164393919520080089569091796875;-0.748255587499393026718053079093806445598602294921875;-0.8930452997856173080748476422741077840328216552734375;-0.3068847913407621863512986237765289843082427978515625;0.5477080755002823320154448083485476672649383544921875;-0.98925761512351118032171370941796340048313140869140625;-0.64119907846262014228244652258581481873989105224609375;-0.41004655161942349383963346554082818329334259033203125;-0.2154503146029320415077989991914364509284496307373046875;-1.275394006992440321113235768279992043972015380859375]
      mask Display: e = 0.06;c1 = [120 150 230]/255;c2 = ([120 150 230]+0)/383;c3 = ([120 150 230]+128)/383;patch([0 1 1 0],[0 0 1 1],c1);patch([0 1 1 1-e 1-e 0+e],[0 0 1 1-e 0+e 0+e],c2);patch([0 0 1 1-e 0+e 0+e],[0 1 1 1-e 1-e 0+e],c3);plot([0 1 1 0 0],[0 0 1 1 0]);disp('weights');
  Mux : Mux  Inputs=15
      mask Display: e = 0.06;c1 = [120 150 230]/255;c2 = ([120 150 230]+0)/383;c3 = ([120 150 230]+128)/383;patch([0 1 1 0],[0 0 1 1],c1);patch([0 1 1 1-e 1-e 0+e],[0 0 1 1-e 0+e 0+e],c2);patch([0 0 1 1-e 0+e 0+e],[0 1 1 1-e 1-e 0+e],c3);plot([0 1 1 0 0],[0 0 1 1 0]);disp('Mux');
  dotprod{1..15} (15 alike) : neural/Weight Functions/dotprod
  "lz{4,3}" : Outport
      mask Display: e = 0.06;c1 = [120 230 180]/255;c2 = ([120 230 180]+0)/(256+128);c3 = ([120 230 180]+128)/(256+128);patch([0 1 1 0],[0 0 1 1],c1);patch([0 1 1 1-e 1-e 0+e],[0 0 1 1-e 0+e 0+e],c2);patch([0 0 1 1-e 0+e 0+e],[0 1 1 1-e 1-e 0+e],c3);plot([0 1 1 0 0],[0 0 1 1 0]);
  wires:
  Mux/1 -> "lz{4,3}"/1
  dotprod15/1 -> Mux/15
  "IW{4,3}(15,:)'"/1 -> dotprod15/1
  dotprod14/1 -> Mux/14
  "IW{4,3}(14,:)'"/1 -> dotprod14/1
  dotprod13/1 -> Mux/13
  "IW{4,3}(13,:)'"/1 -> dotprod13/1
  dotprod12/1 -> Mux/12
  "IW{4,3}(12,:)'"/1 -> dotprod12/1
  dotprod11/1 -> Mux/11
  "IW{4,3}(11,:)'"/1 -> dotprod11/1
  dotprod10/1 -> Mux/10
  "IW{4,3}(10,:)'"/1 -> dotprod10/1
  dotprod9/1 -> Mux/9
  "IW{4,3}(9,:)'"/1 -> dotprod9/1
  dotprod8/1 -> Mux/8
  "IW{4,3}(8,:)'"/1 -> dotprod8/1
  dotprod7/1 -> Mux/7
  "IW{4,3}(7,:)'"/1 -> dotprod7/1
  dotprod6/1 -> Mux/6
  "IW{4,3}(6,:)'"/1 -> dotprod6/1
  dotprod5/1 -> Mux/5
  "IW{4,3}(5,:)'"/1 -> dotprod5/1
  dotprod4/1 -> Mux/4
  "IW{4,3}(4,:)'"/1 -> dotprod4/1
  dotprod3/1 -> Mux/3
  "IW{4,3}(3,:)'"/1 -> dotprod3/1
  dotprod2/1 -> Mux/2
  "IW{4,3}(2,:)'"/1 -> dotprod2/1
  dotprod1/1 -> Mux/1
  "ad{4,3}"/1 -> dotprod15/2, dotprod14/2, dotprod13/2, dotprod12/2, dotprod11/2, dotprod10/2, dotprod9/2, dotprod8/2, dotprod7/2, dotprod6/2, dotprod5/2, dotprod4/2, dotprod3/2, dotprod2/2, dotprod1/2
  "IW{4,3}(1,:)'"/1 -> dotprod1/1

== system AFC_FFNN_trainbfg_15_15_15_15_Nor_July_15_RepFast/Air Fuel Control Model 1/Feed-Forward Neural Network/Layer 5/Delays 1 ==
  "p{5}" : Inport  PortDimensions=15
      mask Display: e = 0.06;c1 = [120 230 180]/255;c2 = ([120 230 180]+0)/(256+128);c3 = ([120 230 180]+128)/(256+128);patch([0 1 1 0],[0 0 1 1],c1);patch([0 1 1 1-e 1-e 0+e],[0 0 1 1-e 0+e 0+e],c2);patch([0 0 1 1-e 0+e 0+e],[0 1 1 1-e 1-e 0+e],c3);plot([0 1 1 0 0],[0 0 1 1 0]);
  mux : Mux  Inputs=1
      mask Display: e = 0.06;c1 = [120 150 230]/255;c2 = ([120 150 230]+0)/383;c3 = ([120 150 230]+128)/383;patch([0 1 1 0],[0 0 1 1],c1);patch([0 1 1 1-e 1-e 0+e],[0 0 1 1-e 0+e 0+e],c2);patch([0 0 1 1-e 0+e 0+e],[0 1 1 1-e 1-e 0+e],c3);plot([0 1 1 0 0],[0 0 1 1 0]);disp('Mux')
  "pd{5,4}" : Outport
      mask Display: e = 0.06;c1 = [120 230 180]/255;c2 = ([120 230 180]+0)/(256+128);c3 = ([120 230 180]+128)/(256+128);patch([0 1 1 0],[0 0 1 1],c1);patch([0 1 1 1-e 1-e 0+e],[0 0 1 1-e 0+e 0+e],c2);patch([0 0 1 1-e 0+e 0+e],[0 1 1 1-e 1-e 0+e],c3);plot([0 1 1 0 0],[0 0 1 1 0]);
  wires:
  mux/1 -> "pd{5,4}"/1
  "p{5}"/1 -> mux/1

== system AFC_FFNN_trainbfg_15_15_15_15_Nor_July_15_RepFast/Air Fuel Control Model 1/Feed-Forward Neural Network/Layer 5/LW{5,4} ==
  "ad{5,4}" : Inport  PortDimensions=15
      mask Display: e = 0.06;c1 = [120 230 180]/255;c2 = ([120 230 180]+0)/(256+128);c3 = ([120 230 180]+128)/(256+128);patch([0 1 1 0],[0 0 1 1],c1);patch([0 1 1 1-e 1-e 0+e],[0 0 1 1-e 0+e 0+e],c2);patch([0 0 1 1-e 0+e 0+e],[0 1 1 1-e 1-e 0+e],c3);plot([0 1 1 0 0],[0 0 1 1 0]);
  "IW{5,4}(1,:)'" : Constant  Value=[0.63232546415590906718762198579497635364532470703125;-0.169051723874596770968992132111452519893646240234375;-0.69946240155650063474723765466478653252124786376953125;0.459821670027029227867387817241251468658447265625;0.39674119614733693861552410453441552817821502685546875;-0.9852702587518942234368068966432474553585052490234375;-0.338339474410549456706576165743172168731689453125;0.474516192083134058510296426902641542255878448486328125;0.33806496686015063968255844883969984948635101318359375;0.1484491629542154245147145275041111744940280914306640625;0.229695058132312557308551959067699499428272247314453125;1.7530956139152760187016610871069133281707763671875;0.716214319281081035484248786815442144870758056640625;-0.150907167366728989232882440774119459092617034912109375;0.273084464625173328755636248388327658176422119140625]
      mask Display: e = 0.06;c1 = [120 150 230]/255;c2 = ([120 150 230]+0)/383;c3 = ([120 150 230]+128)/383;patch([0 1 1 0],[0 0 1 1],c1);patch([0 1 1 1-e 1-e 0+e],[0 0 1 1-e 0+e 0+e],c2);patch([0 0 1 1-e 0+e 0+e],[0 1 1 1-e 1-e 0+e],c3);plot([0 1 1 0 0],[0 0 1 1 0]);disp('weights');
  Mux : Mux  Inputs=1
      mask Display: e = 0.06;c1 = [120 150 230]/255;c2 = ([120 150 230]+0)/383;c3 = ([120 150 230]+128)/383;patch([0 1 1 0],[0 0 1 1],c1);patch([0 1 1 1-e 1-e 0+e],[0 0 1 1-e 0+e 0+e],c2);patch([0 0 1 1-e 0+e 0+e],[0 1 1 1-e 1-e 0+e],c3);plot([0 1 1 0 0],[0 0 1 1 0]);disp('Mux');
  dotprod1 : neural/Weight Functions/dotprod
  "lz{5,4}" : Outport
      mask Display: e = 0.06;c1 = [120 230 180]/255;c2 = ([120 230 180]+0)/(256+128);c3 = ([120 230 180]+128)/(256+128);patch([0 1 1 0],[0 0 1 1],c1);patch([0 1 1 1-e 1-e 0+e],[0 0 1 1-e 0+e 0+e],c2);patch([0 0 1 1-e 0+e 0+e],[0 1 1 1-e 1-e 0+e],c3);plot([0 1 1 0 0],[0 0 1 1 0]);
  wires:
  Mux/1 -> "lz{5,4}"/1
  dotprod1/1 -> Mux/1
  "ad{5,4}"/1 -> dotprod1/2
  "IW{5,4}(1,:)'"/1 -> dotprod1/1
